simulink model "Second_order_loop"  (R2025a)
settings: Solver=VariableStepAuto  StartTime=0.0  StopTime=50  RelTol=1e-3
libraries: simulink x2
settings Model: Creator=庞亚宸  LastModifiedBy=庞亚宸

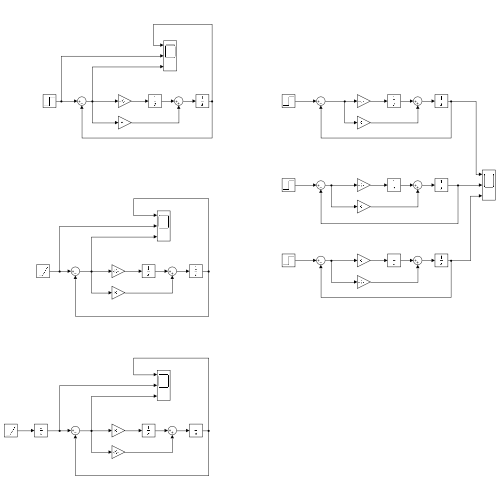
[thumbnail: Simulink's stored preview of the top-level diagram]
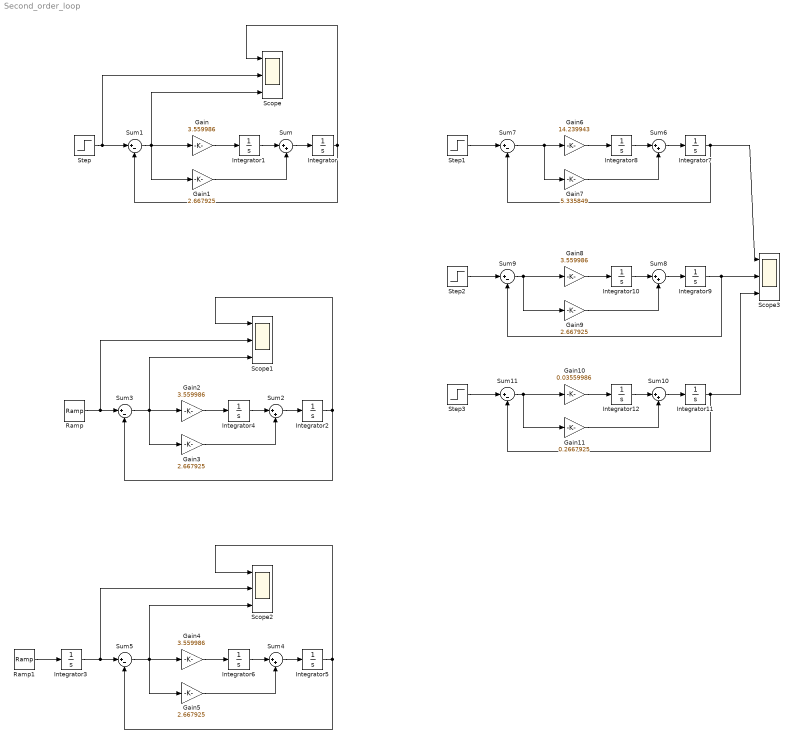
== system Second_order_loop ==
  Gain{,2,4,8} (4 alike) : Gain  Gain=3.559986
  Gain{1,3,5,9} (4 alike) : Gain  Gain=2.667925
  Gain10 : Gain  Gain=0.03559986
  Gain11 : Gain  Gain=0.2667925
  Gain6 : Gain  Gain=14.239943
  Gain7 : Gain  Gain=5.335849
  Integrator{,1..12} (13 alike) : Integrator
  Ramp : simulink/Sources/Ramp  slope=1  start=0  InitialOutput=0
  Ramp1 : simulink/Sources/Ramp  slope=1  start=0  InitialOutput=0
  Scope{,1..3} (4 alike) : Scope  NumInputPorts=3
      Scope settings: ActiveDisplayYMinimum=-0.15090706420541608  ActiveDisplayYMaximum=1.3581635778487451
      Scope1 settings: ActiveDisplayYMinimum=-1.2499998942511912  ActiveDisplayYMaximum=11.249999048260722
      Scope2 settings: ActiveDisplayYMinimum=-6.2148875822732075  ActiveDisplayYMaximum=55.933988240458881  DataLoggingVariableName=ScopeData2
      Scope3 settings: ActiveDisplayYMinimum=-0.15083955126036255  ActiveDisplayYMaximum=1.3575559613432633  DataLoggingVariableName=ScopeData3
  Step{,1..3} (4 alike) : Step  Time=0  SampleTime=0
  Sum{,2,4,6,8,10} (6 alike) : Sum  Inputs=|++
  Sum{1,3,5,7,9,11} (6 alike) : Sum  Inputs=|+-
  wires:
  Sum1/1 -> Scope/3, Gain1/1, Gain/1
  Gain/1 -> Integrator1/1
  Step/1 -> Scope/2, Sum1/1
  Integrator1/1 -> Sum/1
  Sum/1 -> Integrator/1
  Gain1/1 -> Sum/2
  Integrator/1 -> Sum1/2, Scope/1
  Ramp1/1 -> Integrator3/1
  Sum2/1 -> Integrator2/1
  Gain3/1 -> Sum2/2
  Gain2/1 -> Integrator4/1
  Integrator4/1 -> Sum2/1
  Ramp/1 -> Scope1/2, Sum3/1
  Sum3/1 -> Scope1/3, Gain3/1, Gain2/1
  Integrator2/1 -> Sum3/2, Scope1/1
  Sum4/1 -> Integrator5/1
  Gain5/1 -> Sum4/2
  Gain4/1 -> Integrator6/1
  Integrator6/1 -> Sum4/1
  Integrator3/1 -> Scope2/2, Sum5/1
  Sum5/1 -> Scope2/3, Gain5/1, Gain4/1
  Integrator5/1 -> Sum5/2, Scope2/1
  Sum6/1 -> Integrator7/1
  Gain7/1 -> Sum6/2
  Gain6/1 -> Integrator8/1
  Integrator8/1 -> Sum6/1
  Step1/1 -> Sum7/1
  Sum7/1 -> Gain7/1, Gain6/1
  Integrator7/1 -> Sum7/2, Scope3/1
  Sum8/1 -> Integrator9/1
  Sum9/1 -> Gain9/1, Gain8/1
  Step2/1 -> Sum9/1
  Gain8/1 -> Integrator10/1
  Integrator10/1 -> Sum8/1
  Gain9/1 -> Sum8/2
  Integrator9/1 -> Sum9/2, Scope3/2
  Sum10/1 -> Integrator11/1
  Sum11/1 -> Gain11/1, Gain10/1
  Step3/1 -> Sum11/1
  Gain10/1 -> Integrator12/1
  Integrator12/1 -> Sum10/1
  Integrator11/1 -> Scope3/3, Sum11/2
  Gain11/1 -> Sum10/2
